simulink model "CMU_simulink_model"  (R2025b)
settings: Solver=VariableStepAuto  StartTime=0.0  StopTime=1400  RelTol=1e-3
InitFcn:
  | I_desarj = 5;
  | Q_kapasite = 2.5;
  | T_ortam = 25;
  | C_termal = 250;
  | 
  | SOC_1 = 0.85;
  | SOC_2 = 0.72;
  | SOC_3 = 0.80;
  | SOC_4 = 0.82;
  | 
  | SOC_tablo = [0.10 0.20 0.30 0.40 0.50 0.60 0.70 0.80 0.90 1.00];
  | OCV_tablo = [3.69 3.73 3.77 3.81 3.85 3.89 3.94 4.00 4.08 4.20];
  | 
  | R_ic1 = 0.050;
  | R_ic2 = 0.065;
  | R_ic3 = 0.052;
  | R_ic4 = 0.044;
model workspace (MAT data in the model file):
  I_desarj = Simulink.Parameter
  I_desarj.Value = 5
  I_desarj.Complexity = 'real'
  I_desarj.Dimensions = [1 1]
  I_desarj.DataType = 'auto'
libraries: fl_lib x10, nesl_utility x9
settings Model: Creator=Kekai  LastModifiedBy=Kekai

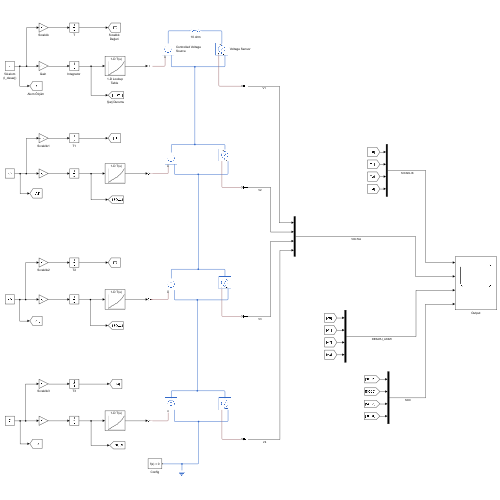
[thumbnail: Simulink's stored preview of the top-level diagram]
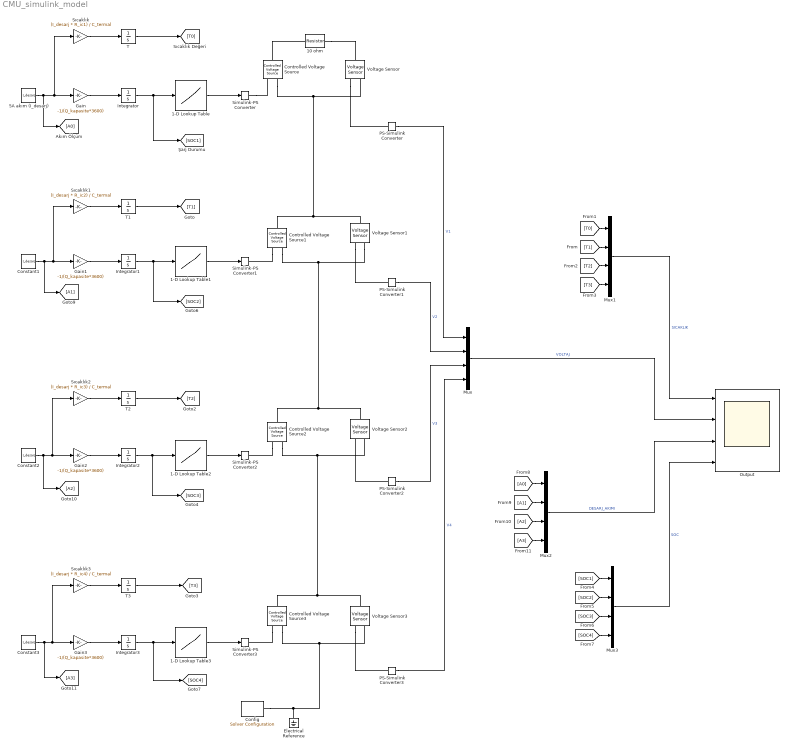
== system CMU_simulink_model ==
  "1-D Lookup Table " : Lookup_n-D  NumberOfTableDimensions=1  BreakpointsForDimension1=SOC_tablo  Table=OCV_tablo  InternalRulePriority=Speed  RndMeth=Simplest
  1-D Lookup Table1 : Lookup_n-D  NumberOfTableDimensions=1  BreakpointsForDimension1=SOC_tablo  Table=OCV_tablo  InternalRulePriority=Speed  RndMeth=Simplest
  1-D Lookup Table2 : Lookup_n-D  NumberOfTableDimensions=1  BreakpointsForDimension1=SOC_tablo  Table=OCV_tablo  InternalRulePriority=Speed  RndMeth=Simplest
  1-D Lookup Table3 : Lookup_n-D  NumberOfTableDimensions=1  BreakpointsForDimension1=SOC_tablo  Table=OCV_tablo  InternalRulePriority=Speed  RndMeth=Simplest
  10 ohm : fl_lib/Electrical/Electrical Elements/Resistor  R=10 Ohm  i_specify=off  i_priority=None  i=0 A  i_nominal_specify=off  i_nominal_value=1  i_nominal_unit=A  v_specify=off  v_priority=None  v=0 V  v_nominal_specify=off  v_nominal_value=1  v_nominal_unit=V
  5A akım (I_desarj) : Constant  Value=I_desarj
  Config : nesl_utility/Solver Configuration  PhysicalDomain=network_engine_domain  SubClassName=solver  LeftPortType=input  RightPortType=generic  Tones=[]  Harmonics=[]  SimulateNoise=off  Profile=off  UseLocalSampling=off  EnableSwitchedLinearOptims=on  FrequencyDomain=off  UseCCode=off  RelTol=0.001  AbsTol=0.001  MinStep=1e-09  ToWorkspace=off  RevertToSquareIcSolve=off  NumHomotopyIterations=100  PhasorMode=off  PhasorModeNumHarmonics=1  ConsistencySolver=NEWTON_XTOL_AFTER_FTOL  IndexReductionMethod=DerivativeReplacement  DoDC=off  ResidualTolerance=1e-09  ConsistencyTolSource=GLOBAL  ConsistencyAbsTol=0.001  ConsistencyRelTol=0.001  ConsistencyTolFactor=0.001  UseLocalSolver=off  LocalSolverChoice=NE_BACKWARD_EULER_ADVANCER  ResolveIndetEquations=on  FunctionEvalNumThread=1  LocalSolverSampleTime=0.001  DoFixedCost=off  MaxNonlinIter=3  MaxModeIter=2  ComputeImpulses=off  ImpulseIterations=2  LinearAlgebra=auto  LinearAlgebraNumThread=0  EquationFormulation=NE_TIME_EF  DelaysMemoryBudget=1024  AutomaticFiltering=on  FilteringTimeConstant=0.001  PartitionStorageMethod=AS_NEEDED  PartitionMemoryBudget=1024  PartitionMethod=ROBUST  MultibodyUseLocalSolver=off  MultibodyLocalSolverChoice=ODE1  MultibodyLocalSolverSampleTime=0.001
  Constant1 : Constant  Value=I_desarj
  Constant2 : Constant  Value=I_desarj
  Constant3 : Constant  Value=I_desarj
  "Controlled Voltage Source " : fl_lib/Electrical/Electrical Sources/Controlled Voltage Source
  Controlled Voltage Source1 : fl_lib/Electrical/Electrical Sources/Controlled Voltage Source
  Controlled Voltage Source2 : fl_lib/Electrical/Electrical Sources/Controlled Voltage Source
  Controlled Voltage Source3 : fl_lib/Electrical/Electrical Sources/Controlled Voltage Source
  Electrical Reference : fl_lib/Electrical/Electrical Elements/Electrical Reference
  "Gain " : Gain  Gain=-1/(Q_kapasite*3600)
  Gain1 : Gain  Gain=-1/(Q_kapasite*3600)
  Gain2 : Gain  Gain=-1/(Q_kapasite*3600)
  Gain3 : Gain  Gain=-1/(Q_kapasite*3600)
  "Integrator " : Integrator  InitialCondition=SOC_1
  Integrator1 : Integrator  InitialCondition=SOC_2
  Integrator2 : Integrator  InitialCondition=SOC_3
  Integrator3 : Integrator  InitialCondition=SOC_4
  Mux{,1..3} (4 alike) : Mux
  Output : Scope  NumInputPorts=4
      settings: ActiveDisplayYMinimum=23.862500000000004  ActiveDisplayYMaximum=35.237499999999969  DataLoggingVariableName=ScopeData8
  PS-Simulink Converter{,1..3} (4 alike) : nesl_utility/PS-Simulink Converter  PhysicalDomain=network_engine_domain  SubClassName=ps_output  LeftPortType=input  RightPortType=output  PseudoPeriodic=off  Frequencies=[]  VectorFormat=inherit  Unit=inherit  AffineConversion=off
  Simulink-PS Converter{,1..3} (4 alike) : nesl_utility/Simulink-PS Converter  PhysicalDomain=network_engine_domain  SubClassName=ps_input  LeftPortType=input  RightPortType=output  PseudoPeriodic=off  Frequencies=[]  NoiseDistribution=none  NoiseParameters=[]  Unit=1  AffineConversion=off  FilteringAndDerivatives=provide  SimscapeFilterOrder=1  InputFilterTimeConstant=0.001  UdotUserProvided=0
  Sıcaklık : Gain  Gain=(I_desarj * R_ic1) / C_termal
  Sıcaklık1 : Gain  Gain=(I_desarj * R_ic2) / C_termal
  Sıcaklık2 : Gain  Gain=(I_desarj * R_ic3) / C_termal
  Sıcaklık3 : Gain  Gain=(I_desarj * R_ic4) / C_termal
  T{,1..3} (4 alike) : Integrator  InitialCondition=T_ortam
  "Voltage Sensor " : fl_lib/Electrical/Electrical Sensors/Voltage Sensor
  Voltage Sensor1 : fl_lib/Electrical/Electrical Sensors/Voltage Sensor
  Voltage Sensor2 : fl_lib/Electrical/Electrical Sensors/Voltage Sensor
  Voltage Sensor3 : fl_lib/Electrical/Electrical Sensors/Voltage Sensor
  wires:
  PS-Simulink Converter3/1 -> Mux/4  "V4"
  PS-Simulink Converter1/1 -> Mux/2  "V2"
  PS-Simulink Converter/1 -> Mux/1  "V1"
  "Integrator "/1 -> [SOC1], "1-D Lookup Table "/1
  "1-D Lookup Table "/1 -> Simulink-PS Converter/1
  1-D Lookup Table1/1 -> Simulink-PS Converter1/1
  Integrator1/1 -> [SOC2], 1-D Lookup Table1/1
  1-D Lookup Table2/1 -> Simulink-PS Converter2/1
  Integrator2/1 -> [SOC3], 1-D Lookup Table2/1
  1-D Lookup Table3/1 -> Simulink-PS Converter3/1
  Integrator3/1 -> [SOC4], 1-D Lookup Table3/1
  5A akım (I_desarj)/1 -> [A0], "Gain "/1, Sıcaklık/1
  "Gain "/1 -> "Integrator "/1
  Constant1/1 -> [A1], Sıcaklık1/1, Gain1/1
  Constant2/1 -> [A2], Sıcaklık2/1, Gain2/1
  Gain1/1 -> Integrator1/1
  Gain2/1 -> Integrator2/1
  Gain3/1 -> Integrator3/1
  Sıcaklık/1 -> T/1
  Mux/1 -> Output/2  "VOLTAJ"
  Mux1/1 -> Output/1  "SICAKLIK"
  Sıcaklık1/1 -> T1/1
  T1/1 -> [T1]
  [T1] -> Mux1/2
  [T0] -> Mux1/1
  T/1 -> [T0]
  Sıcaklık2/1 -> T2/1
  T2/1 -> [T2]
  [T2] -> Mux1/3
  T3/1 -> [T3]
  Sıcaklık3/1 -> T3/1
  Constant3/1 -> [A3], Sıcaklık3/1, Gain3/1
  PS-Simulink Converter2/1 -> Mux/3  "V3"
  [T3] -> Mux1/4
  Mux2/1 -> Output/3  "DESARJ_AKIMI"
  Mux3/1 -> Output/4  "SOC"
  [A0] -> Mux2/1
  [A1] -> Mux2/2
  [SOC2] -> Mux3/2
  [SOC3] -> Mux3/3
  [SOC1] -> Mux3/1
  [SOC4] -> Mux3/4
  [A2] -> Mux2/3
  [A3] -> Mux2/4
  connections:
  Voltage Sensor1/RConn2 -- Controlled Voltage Source1/RConn2 -- Controlled Voltage Source2/LConn1 -- Voltage Sensor2/LConn1
  Voltage Sensor3/LConn1 -- Controlled Voltage Source3/LConn1 -- Voltage Sensor2/RConn2 -- Controlled Voltage Source2/RConn2
  Voltage Sensor1/LConn1 -- Controlled Voltage Source1/LConn1 -- "Controlled Voltage Source "/RConn2 -- "Voltage Sensor "/RConn2
  Config/RConn1 -- Electrical Reference/LConn1 -- Controlled Voltage Source3/RConn2 -- Voltage Sensor3/RConn2
  10 ohm/RConn1 -- "Voltage Sensor "/LConn1
  Voltage Sensor3/RConn1 -- PS-Simulink Converter3/LConn1
  "Voltage Sensor "/RConn1 -- PS-Simulink Converter/LConn1
  Voltage Sensor1/RConn1 -- PS-Simulink Converter1/LConn1
  PS-Simulink Converter2/LConn1 -- Voltage Sensor2/RConn1
  "Controlled Voltage Source "/LConn1 -- 10 ohm/LConn1
  Simulink-PS Converter/RConn1 -- "Controlled Voltage Source "/RConn1
  Controlled Voltage Source1/RConn1 -- Simulink-PS Converter1/RConn1
  Controlled Voltage Source2/RConn1 -- Simulink-PS Converter2/RConn1
  Controlled Voltage Source3/RConn1 -- Simulink-PS Converter3/RConn1
